simulink model "PartD"  (R2021a)
settings: Solver=ode4  StartTime=0.0  StopTime=10  FixedStep=0.0003  RelTol=1e-3
libraries: pid_lib x3
settings Model: Creator=Dimuthu  LastModifiedBy=ASUS
settings SolverCC: AlgebraicLoopSolver=TrustRegion
settings OptimizationCC: LifeSpan=inf
settings DebuggingCC: SFExecutionAtInitializationDiag=none  SFMachineParentedDataDiag=warning  ArithmeticOperatorsInVariantConditions=warning
settings HardwareCC: ProdBitPerSizeT=32  ProdBitPerPtrDiffT=32  ProdWordSize=32  ProdHWDeviceType=Specified
settings SFSimCC: CustomCodeUndefinedFunction=UseInterfaceOnly
settings CodeAppCC: StateflowObjectComments=on

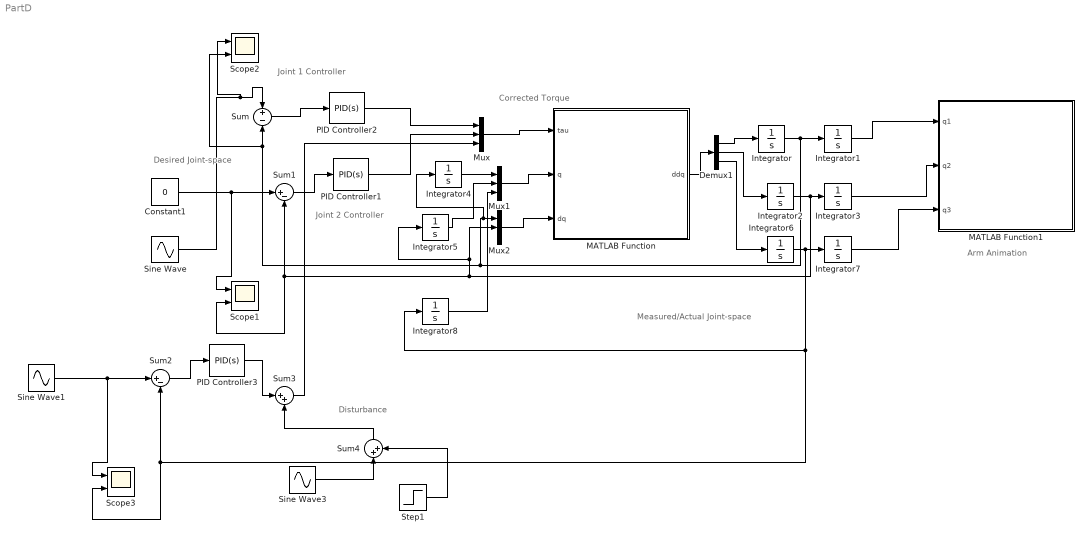
== system PartD ==
  note: Corrected
      | Torque
  note: Desired
      | Joint-space
  note: Measured/Actual Joint-space
  note: Joint 1
      | Controller
  note: Joint 2
      | Controller
  note: Arm Animation
  note: Disturbance
  Constant1 : Constant  Value=0
  Demux1 : Demux  Outputs=3
  Integrator{,1..8} (9 alike) : Integrator
  MATLAB Function : MATLAB Function  TreatAsAtomicUnit=on
  MATLAB Function1 : MATLAB Function  TreatAsAtomicUnit=on
  Mux : Mux  Inputs=3
  Mux1 : Mux  Inputs=3
  Mux2 : Mux  Inputs=3
  PID Controller1 : pid_lib/PID Controller  Controller=PID  Form=Parallel  TimeDomain=Continuous-time  UseExternalTs=off  SampleTime=-1  IntegratorMethod=Forward Euler  FilterMethod=Forward Euler  ControllerParametersSource=internal  P=50  I=50  D=10  UseFilter=on  N=50  TunerSelectOption=Transfer Function Based (PID Tuner App)  InitialConditionSource=internal  InitialConditionForIntegrator=0  InitialConditionForFilter=0  DifferentiatorICPrevScaledInput=0  ExternalReset=none  TrackingMode=off  Kt=1  LimitOutput=off  SatLimitsSource=internal  UpperSaturationLimit=inf  LowerSaturationLimit=-inf  LinearizeAsGain=on  AntiWindupMode=none  Kb=1  POutMin=[]  POutMax=[]  IOutMin=[]  IOutMax=[]  DOutMin=[]  DOutMax=[]  NOutMin=[]  NOutMax=[]  SumOutMin=[]  SumOutMax=[]  SaturationOutMin=[]  SaturationOutMax=[]  PParamMin=[]  PParamMax=[]  IParamMin=[]  IParamMax=[]  DParamMin=[]  DParamMax=[]  NParamMin=[]  NParamMax=[]  KbParamMin=[]  KbParamMax=[]  KtParamMin=[]  KtParamMax=[]  KbOutMin=[]  KbOutMax=[]  KtOutMin=[]  KtOutMax=[]  IntegratorOutMin=[]  IntegratorOutMax=[]  FilterOutMin=[]  FilterOutMax=[]  SumI1OutMin=[]  SumI1OutMax=[]  SumI2OutMin=[]  SumI2OutMax=[]  SumI3OutMin=[]  SumI3OutMax=[]  SumI4OutMin=[]  SumI4OutMax=[]  SumDOutMin=[]  SumDOutMax=[]  DifferentiatorOutMin=[]  DifferentiatorOutMax=[]  FilterDiffOutCoefMin=[]  FilterDiffOutCoefMax=[]  ReciprocalOutMin=[]  ReciprocalOutMax=[]  SumDenOutMin=[]  SumDenOutMax=[]  SumNumOutMin=[]  SumNumOutMax=[]  DivideOutMin=[]  DivideOutMax=[]  UdiffTsProdOutMin=[]  UdiffTsProdOutMax=[]  NTsProdOutMin=[]  NTsProdOutMax=[]  UintegralTsProdOutMin=[]  UintegralTsProdOutMax=[]  UngainTsProdOutMin=[]  UngainTsProdOutMax=[]  IntegratorContinuousStateAttributes=''  IntegratorStateMustResolveToSignalObject=off  IntegratorRTWStateStorageClass=Auto  FilterContinuousStateAttributes=''  FilterStateMustResolveToSignalObject=off  FilterRTWStateStorageClass=Auto  ParallelPVariant=InternalParameters  IdealPVariant=Disabled  IVariant=InternalParameters  DVariant=InternalParameters  IntegratorVariant=Continuous  SatVariant=Disabled  AWVariant=Passthrough  PCopyVariant=Disabled  TRVariant=Disabled  FdbkBlocksVariant=Forward  IdealPFdbkVariant=Disabled  SatFdbkVariant=Disabled  DerivativeFilterVariant=ContFilter  NVariant=InternalParameters  NCopyVariant=Disabled  FilterICVariant=InternalICsFilter  IntegratorICVariant=InternalICs  ExternalResetVariant=Disabled  TRSumVariant=Passthrough  SumFdbkVariant=Disabled  SumVariant=Sum_PID  TsampFilterVariant=InternalTs  TsampNgainVariant=Passthrough  TsampIntegralVariant=Passthrough  ExternalSaturationOutDataTypeStr=Inherit: Same as second input
  PID Controller2 : pid_lib/PID Controller  Controller=PID  Form=Parallel  TimeDomain=Continuous-time  UseExternalTs=off  SampleTime=-1  IntegratorMethod=Forward Euler  FilterMethod=Forward Euler  ControllerParametersSource=internal  P=50  I=50  D=10  UseFilter=on  N=50  TunerSelectOption=Transfer Function Based (PID Tuner App)  InitialConditionSource=internal  InitialConditionForIntegrator=0  InitialConditionForFilter=0  DifferentiatorICPrevScaledInput=0  ExternalReset=none  TrackingMode=off  Kt=1  LimitOutput=off  SatLimitsSource=internal  UpperSaturationLimit=inf  LowerSaturationLimit=-inf  LinearizeAsGain=on  AntiWindupMode=none  Kb=1  POutMin=[]  POutMax=[]  IOutMin=[]  IOutMax=[]  DOutMin=[]  DOutMax=[]  NOutMin=[]  NOutMax=[]  SumOutMin=[]  SumOutMax=[]  SaturationOutMin=[]  SaturationOutMax=[]  PParamMin=[]  PParamMax=[]  IParamMin=[]  IParamMax=[]  DParamMin=[]  DParamMax=[]  NParamMin=[]  NParamMax=[]  KbParamMin=[]  KbParamMax=[]  KtParamMin=[]  KtParamMax=[]  KbOutMin=[]  KbOutMax=[]  KtOutMin=[]  KtOutMax=[]  IntegratorOutMin=[]  IntegratorOutMax=[]  FilterOutMin=[]  FilterOutMax=[]  SumI1OutMin=[]  SumI1OutMax=[]  SumI2OutMin=[]  SumI2OutMax=[]  SumI3OutMin=[]  SumI3OutMax=[]  SumI4OutMin=[]  SumI4OutMax=[]  SumDOutMin=[]  SumDOutMax=[]  DifferentiatorOutMin=[]  DifferentiatorOutMax=[]  FilterDiffOutCoefMin=[]  FilterDiffOutCoefMax=[]  ReciprocalOutMin=[]  ReciprocalOutMax=[]  SumDenOutMin=[]  SumDenOutMax=[]  SumNumOutMin=[]  SumNumOutMax=[]  DivideOutMin=[]  DivideOutMax=[]  UdiffTsProdOutMin=[]  UdiffTsProdOutMax=[]  NTsProdOutMin=[]  NTsProdOutMax=[]  UintegralTsProdOutMin=[]  UintegralTsProdOutMax=[]  UngainTsProdOutMin=[]  UngainTsProdOutMax=[]  IntegratorContinuousStateAttributes=''  IntegratorStateMustResolveToSignalObject=off  IntegratorRTWStateStorageClass=Auto  FilterContinuousStateAttributes=''  FilterStateMustResolveToSignalObject=off  FilterRTWStateStorageClass=Auto  ParallelPVariant=InternalParameters  IdealPVariant=Disabled  IVariant=InternalParameters  DVariant=InternalParameters  IntegratorVariant=Continuous  SatVariant=Disabled  AWVariant=Passthrough  PCopyVariant=Disabled  TRVariant=Disabled  FdbkBlocksVariant=Forward  IdealPFdbkVariant=Disabled  SatFdbkVariant=Disabled  DerivativeFilterVariant=ContFilter  NVariant=InternalParameters  NCopyVariant=Disabled  FilterICVariant=InternalICsFilter  IntegratorICVariant=InternalICs  ExternalResetVariant=Disabled  TRSumVariant=Passthrough  SumFdbkVariant=Disabled  SumVariant=Sum_PID  TsampFilterVariant=InternalTs  TsampNgainVariant=Passthrough  TsampIntegralVariant=Passthrough  ExternalSaturationOutDataTypeStr=Inherit: Same as second input
  PID Controller3 : pid_lib/PID Controller  Controller=PID  Form=Parallel  TimeDomain=Continuous-time  UseExternalTs=off  SampleTime=-1  IntegratorMethod=Forward Euler  FilterMethod=Forward Euler  ControllerParametersSource=internal  P=50  I=50  D=10  UseFilter=on  N=50  TunerSelectOption=Transfer Function Based (PID Tuner App)  InitialConditionSource=internal  InitialConditionForIntegrator=0  InitialConditionForFilter=0  DifferentiatorICPrevScaledInput=0  ExternalReset=none  TrackingMode=off  Kt=1  LimitOutput=off  SatLimitsSource=internal  UpperSaturationLimit=inf  LowerSaturationLimit=-inf  LinearizeAsGain=on  AntiWindupMode=none  Kb=1  POutMin=[]  POutMax=[]  IOutMin=[]  IOutMax=[]  DOutMin=[]  DOutMax=[]  NOutMin=[]  NOutMax=[]  SumOutMin=[]  SumOutMax=[]  SaturationOutMin=[]  SaturationOutMax=[]  PParamMin=[]  PParamMax=[]  IParamMin=[]  IParamMax=[]  DParamMin=[]  DParamMax=[]  NParamMin=[]  NParamMax=[]  KbParamMin=[]  KbParamMax=[]  KtParamMin=[]  KtParamMax=[]  KbOutMin=[]  KbOutMax=[]  KtOutMin=[]  KtOutMax=[]  IntegratorOutMin=[]  IntegratorOutMax=[]  FilterOutMin=[]  FilterOutMax=[]  SumI1OutMin=[]  SumI1OutMax=[]  SumI2OutMin=[]  SumI2OutMax=[]  SumI3OutMin=[]  SumI3OutMax=[]  SumI4OutMin=[]  SumI4OutMax=[]  SumDOutMin=[]  SumDOutMax=[]  DifferentiatorOutMin=[]  DifferentiatorOutMax=[]  FilterDiffOutCoefMin=[]  FilterDiffOutCoefMax=[]  ReciprocalOutMin=[]  ReciprocalOutMax=[]  SumDenOutMin=[]  SumDenOutMax=[]  SumNumOutMin=[]  SumNumOutMax=[]  DivideOutMin=[]  DivideOutMax=[]  UdiffTsProdOutMin=[]  UdiffTsProdOutMax=[]  NTsProdOutMin=[]  NTsProdOutMax=[]  UintegralTsProdOutMin=[]  UintegralTsProdOutMax=[]  UngainTsProdOutMin=[]  UngainTsProdOutMax=[]  IntegratorContinuousStateAttributes=''  IntegratorStateMustResolveToSignalObject=off  IntegratorRTWStateStorageClass=Auto  FilterContinuousStateAttributes=''  FilterStateMustResolveToSignalObject=off  FilterRTWStateStorageClass=Auto  ParallelPVariant=InternalParameters  IdealPVariant=Disabled  IVariant=InternalParameters  DVariant=InternalParameters  IntegratorVariant=Continuous  SatVariant=Disabled  AWVariant=Passthrough  PCopyVariant=Disabled  TRVariant=Disabled  FdbkBlocksVariant=Forward  IdealPFdbkVariant=Disabled  SatFdbkVariant=Disabled  DerivativeFilterVariant=ContFilter  NVariant=InternalParameters  NCopyVariant=Disabled  FilterICVariant=InternalICsFilter  IntegratorICVariant=InternalICs  ExternalResetVariant=Disabled  TRSumVariant=Passthrough  SumFdbkVariant=Disabled  SumVariant=Sum_PID  TsampFilterVariant=InternalTs  TsampNgainVariant=Passthrough  TsampIntegralVariant=Passthrough  ExternalSaturationOutDataTypeStr=Inherit: Same as second input
  Scope1 : Scope  NumInputPorts=2
  Scope2 : Scope  NumInputPorts=2
  Scope3 : Scope  NumInputPorts=2
  Sine Wave : Sin  Amplitude=20*pi/180  Frequency=0.628  SampleTime=0
  Sine Wave1 : Sin  Amplitude=18*pi/180  Frequency=0.628  Phase=pi/6  SampleTime=0
  Sine Wave3 : Sin  Amplitude=10  Frequency=2  SampleTime=0
  Step1 : Step  Time=3  After=10  SampleTime=0
  Sum : Sum  Inputs=+-
  Sum1 : Sum  Inputs=|+-
  Sum2 : Sum  Inputs=|+-
  Sum3 : Sum  Inputs=|++
  Sum4 : Sum  Inputs=|++
  wires:
  Sum1/1 -> PID Controller1/1
  Integrator1/1 -> MATLAB Function1/1(q1)
  Integrator2/1 -> Sum1/2, Scope1/2, Mux2/2, Integrator5/1, Integrator3/1
  Demux1/1 -> Integrator/1
  Integrator/1 -> Sum/2, Scope2/2, Integrator4/1, Mux2/1, Integrator1/1
  Demux1/2 -> Integrator2/1
  Integrator3/1 -> MATLAB Function1/2(q2)
  Sum/1 -> PID Controller2/1
  PID Controller1/1 -> Mux/2
  PID Controller2/1 -> Mux/1
  Constant1/1 -> Scope1/1, Sum1/1
  Mux2/1 -> MATLAB Function/3(dq)
  Mux1/1 -> MATLAB Function/2(q)
  Mux/1 -> MATLAB Function/1(tau)
  MATLAB Function/1(ddq) -> Demux1/1
  Integrator4/1 -> Mux1/1
  Integrator5/1 -> Mux1/2
  Sine Wave/1 -> Scope2/1, Sum/1
  Sum2/1 -> PID Controller3/1
  Integrator6/1 -> Integrator7/1, Integrator8/1, Sum2/2, Scope3/2
  Sine Wave1/1 -> Scope3/1, Sum2/1
  Demux1/3 -> Integrator6/1
  Integrator7/1 -> MATLAB Function1/3(q3)
  Integrator8/1 -> Mux1/3
  Sum4/1 -> Sum3/2
  Step1/1 -> Sum4/2
  Sine Wave3/1 -> Sum4/1
  PID Controller3/1 -> Sum3/1
  Sum3/1 -> Mux/3

== matlab function PartD/MATLAB Function1 ==
  settings: updateMethod=DISCRETE
  data: q1 input double size=1; q2 input double size=1; q3 input
function DrawArm(q1, q2,q3)
%#codegen

% Link lengths
l1 = 1.0;
l2 = 1.0;

% Forward kinematics
x1 = l1 * cos(q1);
y1 = l1 * sin(q1);
x2 = x1 + l2 * cos(q1 + q2);
y2 = y1 + l2 * sin(q1 + q2);

% Persistent variables
persistent h1 h2 base initialized
if isempty(initialized)
    figure(1); clf;
    axis equal; axis([-2.2 2.2 -2.2 2.2]);
    grid on; hold on;
    base = plot(0, 0, 'ko', 'MarkerSize', 6, 'MarkerFaceColor', 'k');
    h1 = plot([0, x1], [0, y1], 'r-', 'LineWidth', 5);
    h2 = plot([x1, x2], [y1, y2], 'b-', 'LineWidth', 5);
    initialized = true;
else
    set(h1, 'XData', [0, x1], 'YData', [0, y1]);
    set(h2, 'XData', [x1, x2], 'YData', [y1, y2]);
end

drawnow;

== matlab function PartD/MATLAB Function ==
  data: tau input double size=[3,1]; ddq output double size=[3,1]; q input double size=[3,1]; dq input double size=[3,1]
function ddq = RobotDynamics(tau, q, dq)
% Parameters
m1 = 1; m2 = 1; m3 = 1;
l1 = 1; l2 = 1; l3 = 1;
g = 9.81;

% Center of mass at midpoints
lc1 = l1 / 2;
lc2 = l2 / 2;
lc3 = l3 / 2;

% Moments of inertia (assuming rod rotating about one end)
I1 = m1 * lc1^2;
I2 = m2 * lc2^2;
I3 = m3 * lc3^2;

% Inertia matrix M(q) — with midpoint CoMs
M11 = I1 + I2 + I3 + ...
      m2*(l1^2 + 2*l1*lc2*cos(q(2))) + ...
      m3*(l1^2 + l2^2 + lc3^2 + ...
      2*l1*l2*cos(q(2)) + 2*l1*lc3*cos(q(2)+q(3)) + 2*l2*lc3*cos(q(3)));

M12 = I2 + I3 + ...
      m2*(lc2^2 + l1*lc2*cos(q(2))) + ...
      m3*(l2^2 + lc3^2 + l1*l2*cos(q(2)) + l1*lc3*cos(q(2)+q(3)) + 2*l2*lc3*cos(q(3)));

M13 = I3 + ...
      m3*(lc3^2 + l1*lc3*cos(q(2)+q(3)) + l2*lc3*cos(q(3)));

M21 = M12;
M22 = I2 + I3 + ...
      m2*lc2^2 + ...
      m3*(l2^2 + 2*l2*lc3*cos(q(3)) + lc3^2);

M23 = I3 + m3*(lc3^2 + l2*lc3*cos(q(3)));

M31 = M13;
M32 = M23;
M33 = I3 + m3*lc3^2;

M = [M11 M12 M13; M21 M22 M23; M31 M32 M33];

% Coriolis and Centripetal matrix C(q,dq)
h = -m2*l1*lc2*sin(q(2)) - m3*l1*l2*sin(q(2));
d = -m3*l2*lc3*sin(q(3));
e = -m3*l1*lc3*sin(q(2)+q(3));

C11 = h*dq(2) + (h + d)*dq(3);
C12 = h*(dq(1) + dq(2)) + d*dq(3);
C13 = (d + e)*(dq(1) + dq(2) + dq(3));
C21 = -h*dq(1);
C22 = d*dq(3);
C23 = d*(dq(1) + dq(2) + dq(3));
C31 = -e*dq(1);
C32 = -d*dq(2);
C33 = 0;

C = [C11 C12 C13; C21 C22 C23; C31 C32 C33];

% Gravity vector G(q) — with CoM at midpoints
G1 = m1*lc1*g*cos(q(1)) + ...
     m2*(l1*g*cos(q(1)) + lc2*g*cos(q(1)+q(2))) + ...
     m3*(l1*g*cos(q(1)) + l2*g*cos(q(1)+q(2)) + lc3*g*cos(q(1)+q(2)+q(3)));

G2 = m2*lc2*g*cos(q(1)+q(2)) + ...
     m3*(l2*g*cos(q(1)+q(2)) + lc3*g*cos(q(1)+q(2)+q(3)));

G3 = m3*lc3*g*cos(q(1)+q(2)+q(3));

G = [G1; G2; G3];

% Compute joint accelerations
ddq = M \ (tau - C*dq - G);

% Optional safety check
assert(isequal(size(ddq), [3 1]), 'Output ddq must be 3x1');
end
